simulink model "FOC_physical_2"  (R2024b)
settings: Solver=FixedStepAuto  StartTime=0.0  StopTime=3  FixedStep=1e-5  RelTol=1e-3
undefined symbols (not defined in the file): Down, GPTRIP1SEL, Ki_current, Ki_q, Ki_s, Ki_speed, Kp_current, Kp_q, Kp_s, Kp_speed, lambda, lamdaM, Ld, Ls, ma, P, Rs, T_max, T_period, Ts, TZ1, Up, Vdc
libraries: simulink x8, spsIGBTDiodeLib x6, spsCurrentMeasurementLib x3, eeStairGenerator x3, nesl_utility x2, spsDCVoltageSourceLib x1, spsPermanentMagnetSynchronousMachineLib x1, c2802xlib x1, spsThreePhaseVIMeasurementLib x1, spsVoltageMeasurementLib x1, sps_lib x1
(part 2 of 2)

== matlab function FOC_physical_2/SVPWM/Sector detection ==
  data: u input; S output
function S = fcn(u)

u = (180/pi)* u;

if(u < 60 && u >= 0)
    u = 1;
elseif(u < 120 && u >= 60)
    u = 2;
elseif(u < 180 && u >= 120)
    u = 3;
elseif(u < -120 && u >= -180)
u = 4;
elseif(u < -60 && u >= -120)
u = 5;
elseif(u < 0 && u >= -60)
u = 6;
else
    u = 0;
end
S = u;

== matlab function FOC_physical_2/SVPWM Technique/Sector Detector ==
  data: u input; S output
function S = fcn(u)

  u= 180/(pi)*u ; % rad to degree
  
if (u>=0)&&(u<60)
  u = 1  ; 
elseif (u>=60)&&(u<120)
  u = 2  ;  
elseif (u>=120)&&(u<180)
  u = 3  ;  
elseif (u>=-180)&&(u<-120)
  u = 4  ;
elseif (u>=-120)&&(u<-60)
  u = 5  ;
elseif (u>=-60)&&(u<0)
  u = 6  ;
else
  u=0 ; 
end

S = u;

== matlab function FOC_physical_2/SVPWM Technique/Step 3- Determine the switching time of each transistor (S1 to S6) /Sector detection1 ==
  data: s input; u input; Ts1 output; Ts3 output; v input; w input; g input; Ts5 output
function [Ts1,Ts3,Ts5] = fcn(s,u,v,w,g)

switch s 
  
 case 1 
  Ts1 = u ; 
  Ts3 = v ;
  Ts5 = w ;
 case 2 
  Ts1 = g ; 
  Ts3 = u ; 
  Ts5 = w ;
 case 3 
  Ts1 = w ;
  Ts3 = u ; 
  Ts5 = v ; 
 case 4 
  Ts1 = w ;
  Ts3 = g ; 
  Ts5 = u ;
 case 5 
  Ts1 = v ;
  Ts3 = w ; 
  Ts5 = u ;
 case 6 
  Ts1 = u ;
  Ts3 = w ; 
  Ts5 = g ;
 otherwise 
 Ts1 = 0 ; 
 Ts3 = 0 ;
 Ts5 = 0 ;
 end 

end
